simulink model "IO_FBL_control"  (R2025b)
settings: Solver=VariableStepAuto  StartTime=0.0  StopTime=50.0  RelTol=1e-3
libraries: simulink x2, slpidlib x1
settings Model: Creator=feder  LastModifiedBy=feder

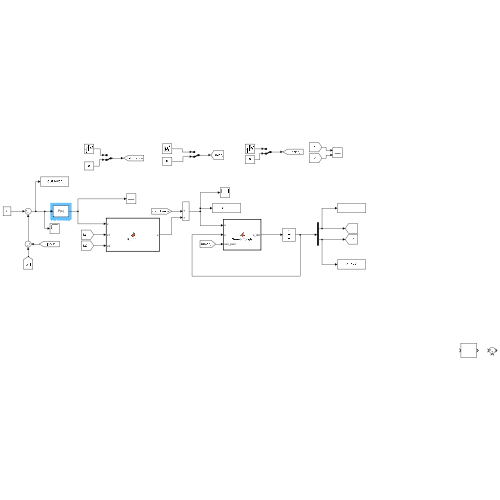
[thumbnail: Simulink's stored preview of the top-level diagram]
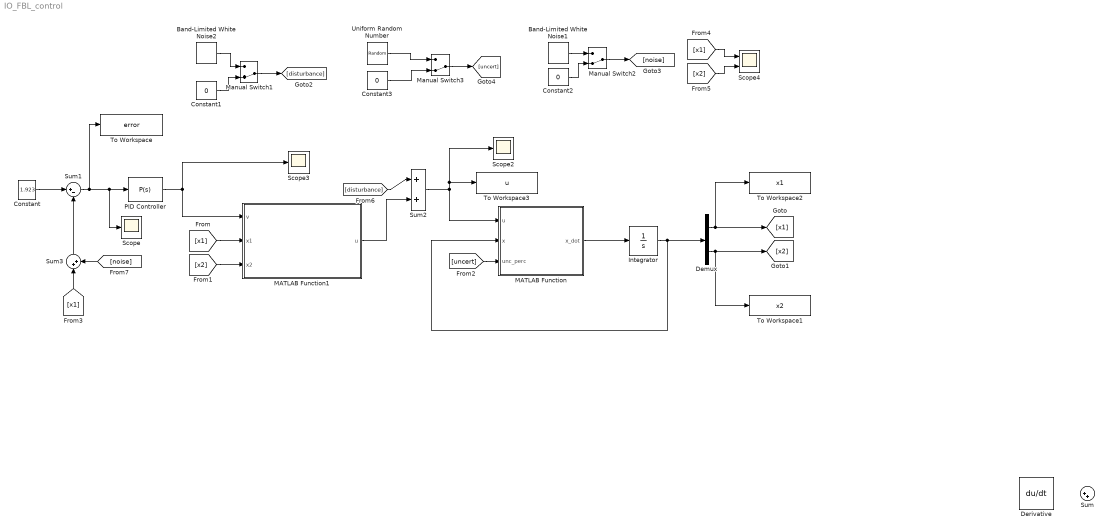
== system IO_FBL_control ==
  Band-Limited White Noise1 : simulink/Sources/Band-Limited White Noise  Cov=[0.001]  Ts=0.01  seed=[23341]
  Band-Limited White Noise2 : simulink/Sources/Band-Limited White Noise  Cov=[0.2]  Ts=0.2  seed=[23341]
  Constant : Constant  Value=1.923
  Constant1 : Constant  Value=0
  Constant2 : Constant  Value=0
  Constant3 : Constant  Value=0
  Demux : Demux  Outputs=2
  Derivative : Derivative
  Integrator : Integrator  InitialCondition=[0.127;7.872]
  MATLAB Function : MATLAB Function  TreatAsAtomicUnit=on
  MATLAB Function1 : MATLAB Function  TreatAsAtomicUnit=on
  Manual Switch1 : ManualSwitch  CurrentSetting=0
  Manual Switch2 : ManualSwitch  CurrentSetting=0
  Manual Switch3 : ManualSwitch  CurrentSetting=0
  PID Controller : slpidlib/PID Controller  Controller=P  Form=Parallel  TimeDomain=Continuous-time  UseExternalTs=off  SampleTime=-1  IntegratorMethod=Forward Euler  FilterMethod=Forward Euler  ControllerParametersSource=internal  P=0.5  I=100  UseKiTs=on  D=2000  UseExternalDerivativeSource=off  N=100  UseFilter=on  TunerSelectOption=Transfer Function Based (PID Tuner App)  InitialConditionSource=internal  InitialConditionForIntegrator=0  InitialConditionForFilter=0  DifferentiatorICPrevScaledInput=0  ExternalReset=none  TrackingMode=off  Kt=1  LimitOutput=off  SatLimitsSource=internal  UpperSaturationLimit=80  LowerSaturationLimit=-10  LinearizeAsGain=on  AntiWindupMode=none  Kb=1  LimitIntegrator=off  UpperIntegratorSaturationLimit=inf  LowerIntegratorSaturationLimit=-inf  POutMin=[]  POutMax=[]  IOutMin=[]  IOutMax=[]  DOutMin=[]  DOutMax=[]  NOutMin=[]  NOutMax=[]  SumOutMin=[]  SumOutMax=[]  SaturationOutMin=[]  SaturationOutMax=[]  PParamMin=[]  PParamMax=[]  IParamMin=[]  IParamMax=[]  DParamMin=[]  DParamMax=[]  NParamMin=[]  NParamMax=[]  KbParamMin=[]  KbParamMax=[]  KtParamMin=[]  KtParamMax=[]  KbOutMin=[]  KbOutMax=[]  KtOutMin=[]  KtOutMax=[]  IntegratorOutMin=[]  IntegratorOutMax=[]  FilterOutMin=[]  FilterOutMax=[]  SumI1OutMin=[]  SumI1OutMax=[]  SumI2OutMin=[]  SumI2OutMax=[]  SumI3OutMin=[]  SumI3OutMax=[]  SumI4OutMin=[]  SumI4OutMax=[]  SumDOutMin=[]  SumDOutMax=[]  DifferentiatorOutMin=[]  DifferentiatorOutMax=[]  FilterDiffOutCoefMin=[]  FilterDiffOutCoefMax=[]  ReciprocalOutMin=[]  ReciprocalOutMax=[]  SumDenOutMin=[]  SumDenOutMax=[]  SumNumOutMin=[]  SumNumOutMax=[]  DivideOutMin=[]  DivideOutMax=[]  UdiffTsProdOutMin=[]  UdiffTsProdOutMax=[]  NTsProdOutMin=[]  NTsProdOutMax=[]  UintegralTsProdOutMin=[]  UintegralTsProdOutMax=[]  UngainTsProdOutMin=[]  UngainTsProdOutMax=[]  ClampingZeroOutDataTypeStr=Inherit: Inherit via back propagation  ClampingZeroOutMin=[]  ClampingZeroOutMax=[]  FilterDenConstantOutDataTypeStr=Inherit: Inherit via back propagation  FilterDenConstantOutMin=[]  FilterDenConstantOutMax=[]  PCopyOutDataTypeStr=Inherit: Inherit via back propagation  PCopyOutMin=[]  PCopyOutMax=[]  NCopyOutDataTypeStr=Inherit: Inherit via back propagation  NCopyOutMin=[]  NCopyOutMax=[]  IntegratorContinuousStateAttributes=''  IntegratorStateMustResolveToSignalObject=off  IntegratorRTWStateStorageClass=Auto  FilterContinuousStateAttributes=''  FilterStateMustResolveToSignalObject=off  FilterRTWStateStorageClass=Auto  ParallelPVariant=InternalParameters  IdealPVariant=Disabled  IVariant=Disabled  DVariant=Disabled  IntegratorVariant=Disabled  SatVariant=Disabled  AWVariant=Disabled  PCopyVariant=Disabled  TRVariant=Disabled  FdbkBlocksVariant=Forward  IdealPFdbkVariant=Disabled  SatFdbkVariant=Disabled  DerivativeFilterVariant=Disabled  NVariant=Disabled  NCopyVariant=Disabled_SignalSpec  FilterICVariant=Disabled  IntegratorICVariant=Disabled  ExternalResetVariant=Disabled  TRSumVariant=Passthrough  SumFdbkVariant=Disabled  SumVariant=Passthrough_P  TsampFilterVariant=InternalTs  TsampNgainVariant=Passthrough  TsampIntegralVariant=Disabled_SignalSpec  ExternalSaturationOutDataTypeStr=Inherit: Same as second input  DerivativeSourceVariant=Disabled  PreIntVariant=InternalPreInt
  Scope : Scope
      settings: ActiveDisplayYMinimum=-1  ActiveDisplayYMaximum=1
  Scope2 : Scope
      settings: ActiveDisplayYMinimum=-1  ActiveDisplayYMaximum=1  DataLoggingVariableName=ScopeData2
  Scope3 : Scope
      settings: ActiveDisplayYMinimum=-1  ActiveDisplayYMaximum=1  DataLoggingVariableName=ScopeData3
  Scope4 : Scope  NumInputPorts=2
      settings: ActiveDisplayYMinimum=-0.097499999996850634  ActiveDisplayYMaximum=2.1474999999716564  DataLoggingVariableName=ScopeData4
  Sum : Sum  Inputs=|++
  Sum1 : Sum  Inputs=|+-
  Sum2 : Sum  Inputs=|++
  Sum3 : Sum  Inputs=|++
  To Workspace : ToWorkspace  VariableName=error  SaveFormat=Timeseries  SampleTime=-1
  To Workspace1 : ToWorkspace  VariableName=x2  SaveFormat=Timeseries  SampleTime=-1
  To Workspace2 : ToWorkspace  VariableName=x1  SaveFormat=Timeseries  SampleTime=-1
  To Workspace3 : ToWorkspace  VariableName=u  SaveFormat=Timeseries  SampleTime=-1
  Uniform Random Number : UniformRandomNumber  Minimum=-0.3  Maximum=0.3  SampleTime=1e6  VectorParams1D=off
  wires:
  MATLAB Function/1(x_dot) -> Integrator/1
  Integrator/1 -> MATLAB Function/2(x), Demux/1
  Demux/2 -> To Workspace1/1, [x2]
  Demux/1 -> To Workspace2/1, [x1]
  [x1] -> MATLAB Function1/2(x1)
  [x2] -> MATLAB Function1/3(x2)
  Sum1/1 -> To Workspace/1, Scope/1, PID Controller/1
  Constant1/1 -> Manual Switch1/2
  Constant3/1 -> Manual Switch3/2
  Band-Limited White Noise1/1 -> Manual Switch2/1
  Constant2/1 -> Manual Switch2/2
  Manual Switch2/1 -> [noise]
  Manual Switch3/1 -> [uncert]
  Uniform Random Number/1 -> Manual Switch3/1
  Manual Switch1/1 -> [disturbance]
  [x1] -> Scope4/1
  PID Controller/1 -> Scope3/1, MATLAB Function1/1(v)
  [disturbance] -> Sum2/1
  MATLAB Function1/1(u) -> Sum2/2
  [x1] -> Sum3/1
  [noise] -> Sum3/2
  Sum3/1 -> Sum1/2
  Constant/1 -> Sum1/1
  [uncert] -> MATLAB Function/3(unc_perc)
  Band-Limited White Noise2/1 -> Manual Switch1/1
  [x2] -> Scope4/2
  Sum2/1 -> MATLAB Function/1(u), Scope2/1, To Workspace3/1

== matlab function IO_FBL_control/MATLAB Function1 ==
  data: v input; x1 input; u output; x2 input
function u = IO_FBL(v, x1, x2)
    alphaY_nom = 10;      
    betaY  = 0.25;         
    betaZ  = 0.25;         
    gammaY = 1;            
    KY     = 1;                
    KZ     = 1;                
    n      = 2;                
   
    HZ = 1 / (1 + (x2 / KZ)^n);   
    HY = 1 / (1 + (x1 / KY)^n);   
    
 
    D  = 1 + betaY*HZ + betaZ*HY;
    
    %  Lie derivatives for y = x1  
    f1 = (alphaY_nom * HZ / D) - gammaY*x1;
    g1 = (HZ / D);
    u = (v - f1) / g1;
end

== matlab function IO_FBL_control/MATLAB Function ==
  data: u input; x_dot output; x input; unc_perc input
function x_dot = GeneticToggle(u, x, unc_perc)

alphaY_nom = 10; % alpha_Y^{nom}
alphaZ = 10; % alpha_Z
betaY = 0.25; % beta_Y
betaZ = 0.25; % beta_Z
gammaY = 1; % gamma_Y
gammaZ = 1; % gamma_Z
KY = 1; % K_Y
KZ = 1; % K_Z
n = 2; % Hill coefficient


x1 = x(1);
x2 = x(2);

alphaY_eff = alphaY_nom * (1 + unc_perc);
alphaY_act = alphaY_eff + u;


HZ = 1 / (1 + (x2 / KZ)^n);
HY = 1 / (1 + (x1 / KY)^n);

%denominatore
D = 1 + betaY*HZ + betaZ*HY;

dx1 = (alphaY_act * HZ / D) - gammaY*x1;
dx2 = (alphaZ * HY / D) - gammaZ*x2;

x_dot = [dx1; dx2];

end
